simulink model "Chap4_5a"  (R2020b)
settings: Solver=VariableStepAuto  StartTime=0.0  StopTime=10.0  RelTol=1e-3
StopFcn:
  | clc;
  | clear all;
  | close all;
  | dat=load('Data.mat','ans');
  | figure
  | plot(dat.ans.time,dat.ans.data(:,1),dat.ans.time,dat.ans.data(:,2),':')
  | legend('Ideal Dirivative','Modified Dirivative')
  | 
  | figure
  | plot(dat.ans.time,dat.ans.data(:,1),dat.ans.time,dat.ans.data(:,3),':')
  | legend('Ideal Dirivative','Real Dirivative')
  | 
  | figure
  | plot(dat.ans.time,dat.ans.data(:,4),'-',dat.ans.time,dat.ans.data(:,1),':')
  | legend('Original Signal','Dirivative Signal')
  | 
  | figure
  | plot(dat.ans.time,dat.ans.data(:,4),'-',dat.ans.time,dat.ans.data(:,5),':')
  | legend('Ideal Signal','Real Signal')
libraries: simulink x2
settings Model: Creator=yiyon  LastModifiedBy=yiyon

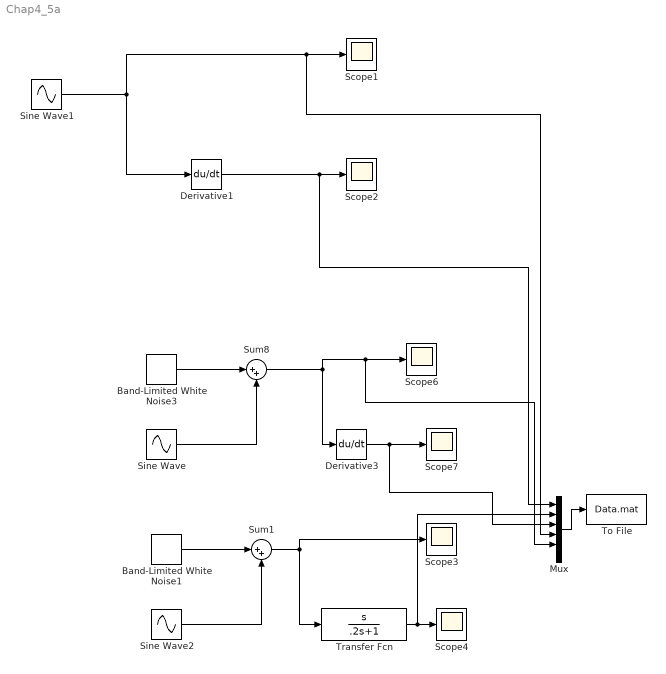
== system Chap4_5a ==
  Band-Limited White Noise1 : simulink/Sources/Band-Limited White Noise  Cov=[0.0001]  Ts=0.01  seed=[23341]
  Band-Limited White Noise3 : simulink/Sources/Band-Limited White Noise  Cov=[0.0001]  Ts=0.01  seed=[23341]
  Derivative1 : Derivative
  Derivative3 : Derivative
  Mux : Mux  Inputs=6
  Scope{1..4,6..7} (6 alike) : Scope
  Sine Wave : Sin  SampleTime=0
  Sine Wave1 : Sin  SampleTime=0
  Sine Wave2 : Sin  SampleTime=0
  Sum1 : Sum  Inputs=|++
  Sum8 : Sum  Inputs=|++
  To File : ToFile  Filename=Data.mat  SaveFormat=Timeseries
  Transfer Fcn : TransferFcn  Numerator=[1 0]  Denominator=[.2 1]
  wires:
  Sine Wave/1 -> Sum8/2
  Sum8/1 -> Mux/5, Scope6/1, Derivative3/1
  Band-Limited White Noise3/1 -> Sum8/1
  Sine Wave1/1 -> Mux/4, Scope1/1, Derivative1/1
  Derivative1/1 -> Mux/1, Scope2/1
  Sum1/1 -> Transfer Fcn/1, Scope3/1
  Band-Limited White Noise1/1 -> Sum1/1
  Sine Wave2/1 -> Sum1/2
  Transfer Fcn/1 -> Mux/2, Scope4/1
  Derivative3/1 -> Mux/3, Scope7/1
  Mux/1 -> To File/1
